simulink model "ESSSimulation"  (R2025a)
settings: Solver=VariableStepAuto  StartTime=0.0  StopTime=1800  RelTol=1e-3
undefined symbols (not defined in the file or in its folder): battery_builder_rtmsupport, gcbh
libraries: nesl_utility x18, P45B_98S30P_Library_lib x14, fl_lib x4, simulink x1, SignalEditorBlockLib x1
(part 3 of 8)

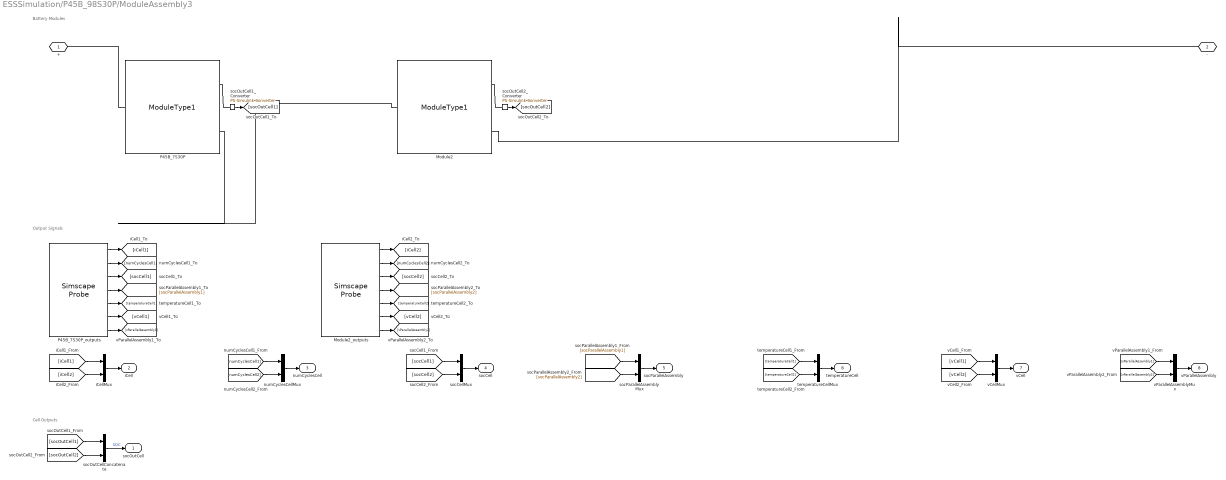
== system ESSSimulation/P45B_98S30P/ModuleAssembly3 ==
  note: Battery Modules
  note: Output Signals
  note: Cell Outputs
  Module2 : P45B_98S30P_Library_lib/Modules/ModuleType1  SOC_vecCell=[0, .01, .02, .03, .04, .05, .06, .07, .08, .09, .1, .11, .12, .13, .14, .15, .16, .17, .18, .19, .2, .21, .22, .23, .24, .25, .26, .27, .28, .29, .3, .31, .32, .33, .34, .35, .36, .37, .38, .39, .4, .41, .42, .43, .44, .45, .46, .47, .48, .49, .5, .51, .52, .53, .54, .55, .56, .57, .58, .59, .6, .61, .62, .63, .64, .65, .66, .67, .68, .69, .7, .71, .72, .73, .74, .75, .76, .77, .78, .79, .8, .81, .82, .83, .84, .85, .86, .87, .88, .89, .9, .91, .92, .93, .94, .95, .96, .97, .98, .99, 1]  T_vecCell=[-40, -30, -20, 0, 23, 45, 60] degC  V0_matCell=[3.17242, 3.17242, 3.17242, 3.17242, 3.17242, 3.17242, 3.17242; 3.18272, 3.18272, 3.18272, 3.18272, 3.18272, 3.18272, 3.18272; 3.19302, 3.19302, 3.19302, 3.19302, 3.19302, 3.19302, 3.19302; 3.20331, 3.20331, 3.20331, 3.20331, 3.20331, 3.20331, 3.20331; 3.21361, 3.21361, 3.21361, 3.21361, 3.21361, 3.21361, 3.21361; 3.22391, 3.22391, 3.22391, 3.22391, 3.22391, 3.22391, 3.22391; 3.23421, 3.23421, 3.23421, 3.23421, 3.23421, 3.23421, 3.23421; 3.24451, 3.24451, 3.24451, 3.24451, 3.24451, 3.24451, 3.24451; 3.25481, 3.25481, 3.25481, 3.25481, 3.25481, 3.25481, 3.25481; 3.2651, 3.2651, 3.2651, 3.2651, 3.2651, 3.2651, 3.2651; 3.2754, 3.2754, 3.2754, 3.2754, 3.2754, 3.2754, 3.2754; 3.2857, 3.2857, 3.2857, 3.2857, 3.2857, 3.2857, 3.2857; 3.296, 3.296, 3.296, 3.296, 3.296, 3.296, 3.296; 3.3063, 3.3063, 3.3063, 3.3063, 3.3063, 3.3063, 3.3063; 3.31659, 3.31659, 3.31659, 3.31659, 3.31659, 3.31659, 3.31659; 3.32689, 3.32689, 3.32689, 3.32689, 3.32689, 3.32689, 3.32689; 3.33719, 3.33719, 3.33719, 3.33719, 3.33719, 3.33719, 3.33719; 3.34749, 3.34749, 3.34749, 3.34749, 3.34749, 3.34749, 3.34749; 3.35779, 3.35779, 3.35779, 3.35779, 3.35779, 3.35779, 3.35779; 3.36809, 3.36809, 3.36809, 3.36809, 3.36809, 3.36809, 3.36809; 3.37838, 3.37838, 3.37838, 3.37838, 3.37838, 3.37838, 3.37838; 3.38868, 3.38868, 3.38868, 3.38868, 3.38868, 3.38868, 3.38868; 3.39898, 3.39898, 3.39898, 3.39898, 3.39898, 3.39898, 3.39898; 3.40928, 3.40928, 3.40928, 3.40928, 3.40928, 3.40928, 3.40928; 3.41958, 3.41958, 3.41958, 3.41958, 3.41958, 3.41958, 3.41958; 3.42988, 3.42988, 3.42988, 3.42988, 3.42988, 3.42988, 3.42988; 3.44017, 3.44017, 3.44017, 3.44017, 3.44017, 3.44017, 3.44017; 3.45047, 3.45047, 3.45047, 3.45047, 3.45047, 3.45047, 3.45047; 3.46077, 3.46077, 3.46077, 3.46077, 3.46077, 3.46077, 3.46077; 3.47107, 3.47107, 3.47107, 3.47107, 3.47107, 3.47107, 3.47107; 3.48137, 3.48137, 3.48137, 3.48137, 3.48137, 3.48137, 3.48137; 3.49166, 3.49166, 3.49166, 3.49166, 3.49166, 3.49166, 3.49166; 3.50196, 3.50196, 3.50196, 3.50196, 3.50196, 3.50196, 3.50196; 3.51226, 3.51226, 3.51226, 3.51226, 3.51226, 3.51226, 3.51226; 3.52256, 3.52256, 3.52256, 3.52256, 3.52256, 3.52256, 3.52256; 3.53286, 3.53286, 3.53286, 3.53286, 3.53286, 3.53286, 3.53286; 3.54316, 3.54316, 3.54316, 3.54316, 3.54316, 3.54316, 3.54316; 3.55345, 3.55345, 3.55345, 3.55345, 3.55345, 3.55345, 3.55345; 3.56375, 3.56375, 3.56375, 3.56375, 3.56375, 3.56375, 3.56375; 3.57405, 3.57405, 3.57405, 3.57405, 3.57405, 3.57405, 3.57405; 3.58435, 3.58435, 3.58435, 3.58435, 3.58435, 3.58435, 3.58435; 3.59465, 3.59465, 3.59465, 3.59465, 3.59465, 3.59465, 3.59465; 3.60495, 3.60495, 3.60495, 3.60495, 3.60495, 3.60495, 3.60495; 3.61524, 3.61524, 3.61524, 3.61524, 3.61524, 3.61524, 3.61524; 3.62554, 3.62554, 3.62554, 3.62554, 3.62554, 3.62554, 3.62554; 3.63584, 3.63584, 3.63584, 3.63584, 3.63584, 3.63584, 3.63584; 3.64614, 3.64614, 3.64614, 3.64614, 3.64614, 3.64614, 3.64614; 3.65644, 3.65644, 3.65644, 3.65644, 3.65644, 3.65644, 3.65644; 3.66673, 3.66673, 3.66673, 3.66673, 3.66673, 3.66673, 3.66673; 3.67703, 3.67703, 3.67703, 3.67703, 3.67703, 3.67703, 3.67703; 3.68733, 3.68733, 3.68733, 3.68733, 3.68733, 3.68733, 3.68733; 3.69763, 3.69763, 3.69763, 3.69763, 3.69763, 3.69763, 3.69763; 3.71041, 3.71041, 3.71041, 3.71041, 3.71041, 3.71041, 3.71041; 3.72113, 3.72113, 3.72113, 3.72113, 3.72113, 3.72113, 3.72113; 3.72997, 3.72997, 3.72997, 3.72997, 3.72997, 3.72997, 3.72997; 3.73882, 3.73882, 3.73882, 3.73882, 3.73882, 3.73882, 3.73882; 3.74912, 3.74912, 3.74912, 3.74912, 3.74912, 3.74912, 3.74912; 3.75936, 3.75936, 3.75936, 3.75936, 3.75936, 3.75936, 3.75936; 3.76951, 3.76951, 3.76951, 3.76951, 3.76951, 3.76951, 3.76951; 3.7791, 3.7791, 3.7791, 3.7791, 3.7791, 3.7791, 3.7791; 3.78865, 3.78865, 3.78865, 3.78865, 3.78865, 3.78865, 3.78865; 3.79787, 3.79787, 3.79787, 3.79787, 3.79787, 3.79787, 3.79787; 3.80709, 3.80709, 3.80709, 3.80709, 3.80709, 3.80709, 3.80709; 3.8161, 3.8161, 3.8161, 3.8161, 3.8161, 3.8161, 3.8161; 3.82509, 3.82509, ...(+2298 chars)] V  V_rangeCell=[2.25, Inf] V  R0_matCell=[.3026, .35142, .34349, .24415, .02095, .15874, .14729; .2941, .33555, .32379, .22614, .01921, .13363, .12249; .28559, .31969, .30408, .20813, .01774, .10853, .10276; .27709, .30382, .28438, .19012, .0166, .09423, .0861; .26858, .28796, .26468, .17211, .01557, .07998, .0748; .26008, .27209, .24498, .1541, .01469, .07024, .06679; .25157, .25623, .22527, .1361, .01398, .06387, .05877; .24307, .24036, .20557, .11861, .01338, .0575, .05275; .23456, .2245, .18587, .10674, .01283, .05113, .04899; .22606, .20863, .16617, .09525, .01239, .04679, .04522; .21755, .19277, .14651, .08799, .01196, .0439, .04145; .20905, .1769, .13098, .08073, .01155, .04101, .03817; .20054, .16103, .11905, .07347, .01116, .03813, .03522; .19204, .14769, .11102, .06895, .01079, .03524, .03228; .18353, .13913, .10517, .06499, .01042, .03235, .02934; .17503, .13157, .09933, .06104, .01007, .02946, .0264; .16653, .1271, .09371, .05708, .00974, .02657, .02345; .15804, .12264, .09094, .05312, .00949, .02417, .02125; .15354, .11817, .08816, .04917, .00924, .02286, .01972; .14976, .11385, .08539, .04748, .009, .02156, .0182; .14598, .11213, .08261, .04617, .00876, .02025, .01667; .14219, .11042, .08103, .04487, .00855, .01894, .01515; .14033, .10871, .08035, .04356, .00843, .01763, .01363; .13876, .10699, .07967, .04225, .00832, .01632, .0121; .13718, .10528, .07899, .04094, .00826, .01501, .01058; .13561, .10357, .07831, .03964, .00825, .0137, .00906; .13404, .10198, .07763, .03833, .00825, .01239, .00753; .13247, .10119, .07695, .03702, .00826, .01108, .0065; .13096, .10039, .07627, .03624, .00827, .00977, .00633; .13043, .0996, .07559, .03615, .00828, .00846, .00617; .1299, .0988, .07491, .03606, .0083, .00774, .006; .12937, .09801, .07423, .03597, .00834, .00779, .00583; .12883, .09721, .07355, .03588, .00838, .00783, .00567; .1283, .09642, .07301, .03579, .00842, .00787, .0055; .12777, .09585, .07296, .0357, .00848, .00792, .00534; .12724, .09584, .07291, .03561, .00855, .00796, .00517; .12675, .09584, .07286, .03552, .00863, .00801, .005; .12643, .09583, .0728, .03543, .00871, .00805, .00484; .12611, .09582, .07275, .03534, .00879, .00809, .00467; .12579, .09582, .0727, .03525, .00887, .00814, .0045; .12547, .09581, .07264, .03526, .00895, .00818, .00434; .12514, .0958, .07259, .03537, .00903, .00823, .00405; .12482, .09579, .07254, .03547, .00911, .00804, .00366; .1245, .09579, .07248, .03558, .00918, .00776, .00327; .12418, .09578, .07243, .03568, .00925, .00748, .00287; .12386, .09577, .07231, .03579, .00931, .0072, .00248; .12354, .09576, .0721, .03589, .00938, .00692, .00209; .12322, .09576, .07189, .036, .00946, .00664, .0017; .12301, .09575, .07168, .03611, .00953, .00636, .00131; .12309, .09574, .07147, .03621, .00961, .00608, .00092; .12318, .09573, .07125, .0363, .00968, .0058, .00053; .12326, .09573, .07104, .03637, .00976, .00552, .00014; .12389, .09628, .07138, .03699, .00991, .00579, .0003; .12407, .09637, .07126, .03715, .01, .0056, .0003; .12383, .09605, .07073, .0369, .01003, .00504, .0003; .12359, .09573, .07019, .03664, .01006, .00503, .0003; .12367, .09573, .06998, .03671, .01013, .00534, .00063; .12375, .09572, .06975, .03677, .01022, .00564, .00094; .1238, .09569, .07006, .0368, .0103, .00593, .00123; .12372, .09554, .07026, .03671, .01037, .00608, .00139; .12364, .09537, .07046, .03661, .01043, .00623, .00155; .12348, .09514, .07058, .03644, .01049, .0063, .00163; .12333, .0949, .07071, .03627, .01055, .00638, .00171; .12312, .09461, .07078, .03605, .01061, .00641, .00175; .12291, .09433, .07085, .03583, .01066, .00643, .00168; .12271, .09404, .07093, .03568, .01072, .00646, .00161; .12275, .09398, .071, .03622, .01077, .00646, .00153; .12316, .09449, .07107, .03677, .01082, .00636, .00145; .12357, .095, .07115, .03731, .01088, .00625, .00137; .12398, .09551, .07151, .03785, .01093, .00614, .00129; .12438, .09601, .07221, .03839, .01099, .00602, .0012; .12486, .09659, .07299, .039, .01105, .00599, .00119; .12548, .09731, .07391, ...(+1578 chars)] Ohm  AHCell=4.493 A*hr  extrapolation_optionCell=simscape.enum.extrapolation.nearest  thermal_massCell=63 J/K  P=30  S=7  iCell_specify=off  iCell_priority=None  iCell=0 A  iCell_nominal_specify=off  iCell_nominal_value=1  iCell_nominal_unit=A  vCell_specify=off  vCell_priority=None  vCell=0 V  vCell_nominal_specify=off  vCell_nominal_value=1  vCell_nominal_unit=V  socCell_specify=off  socCell_priority=High  socCell=1  socCell_nominal_specify=off  socCell_nominal_value=1  socCell_nominal_unit=1  numCyclesCell_specify=off  numCyclesCell_priority=High  numCyclesCell=0  numCyclesCell_nominal_specify=off  numCyclesCell_nominal_value=1  numCyclesCell_nominal_unit=1  temperatureCell_specify=off  temperatureCell_priority=High  temperatureCell=298.15 K  temperatureCell_nominal_specify=off  temperatureCell_nominal_value=1  temperatureCell_nominal_unit=K  vParallelAssembly_specify=off  vParallelAssembly_priority=None  vParallelAssembly=repmat(0, 7, 1) V  vParallelAssembly_nominal_specify=off  vParallelAssembly_nominal_value=1  vParallelAssembly_nominal_unit=V  socParallelAssembly_specify=off  socParallelAssembly_priority=None  socParallelAssembly=repmat(1, 7, 1)  socParallelAssembly_nominal_specify=off  socParallelAssembly_nominal_value=1  socParallelAssembly_nominal_unit=1
      settings: InternalSimscapePortConfiguration="{\"Bottom\":[{\"id\":\"n\",\"label\":\"-\",\"type\":\"foundation.electrical.electrical\"}],\"Left\":[],\"Right\":[{\"id\":\"socOutCell\",\"label\":\"SOC\",\"type\":\"output\"}],\"Top\":[{\"id\":\"p\",\"label\":\"+\",\"type\":\"foundation.electrical.electrical\"}]}"
  Module2_outputs : SimscapeProbe  BoundBlock=63  Variables="{\"iCell\":{\"Probing\":\"ON\"},\"numCyclesCell\":{\"Probing\":\"ON\"},\"socCell\":{\"Probing\":\"ON\"},\"socParallelAssembly\":{\"Probing\":\"ON\"},\"temperatureCell\":{\"Probing\":\"ON\"},\"vCell\":{\"Probing\":\"ON\"},\"vParallelAssembly\":{\"Probing\":\"ON\"}}"
  P45B_7S30P : P45B_98S30P_Library_lib/Modules/ModuleType1  SOC_vecCell=[0, .01, .02, .03, .04, .05, .06, .07, .08, .09, .1, .11, .12, .13, .14, .15, .16, .17, .18, .19, .2, .21, .22, .23, .24, .25, .26, .27, .28, .29, .3, .31, .32, .33, .34, .35, .36, .37, .38, .39, .4, .41, .42, .43, .44, .45, .46, .47, .48, .49, .5, .51, .52, .53, .54, .55, .56, .57, .58, .59, .6, .61, .62, .63, .64, .65, .66, .67, .68, .69, .7, .71, .72, .73, .74, .75, .76, .77, .78, .79, .8, .81, .82, .83, .84, .85, .86, .87, .88, .89, .9, .91, .92, .93, .94, .95, .96, .97, .98, .99, 1]  T_vecCell=[-40, -30, -20, 0, 23, 45, 60] degC  V0_matCell=[3.17242, 3.17242, 3.17242, 3.17242, 3.17242, 3.17242, 3.17242; 3.18272, 3.18272, 3.18272, 3.18272, 3.18272, 3.18272, 3.18272; 3.19302, 3.19302, 3.19302, 3.19302, 3.19302, 3.19302, 3.19302; 3.20331, 3.20331, 3.20331, 3.20331, 3.20331, 3.20331, 3.20331; 3.21361, 3.21361, 3.21361, 3.21361, 3.21361, 3.21361, 3.21361; 3.22391, 3.22391, 3.22391, 3.22391, 3.22391, 3.22391, 3.22391; 3.23421, 3.23421, 3.23421, 3.23421, 3.23421, 3.23421, 3.23421; 3.24451, 3.24451, 3.24451, 3.24451, 3.24451, 3.24451, 3.24451; 3.25481, 3.25481, 3.25481, 3.25481, 3.25481, 3.25481, 3.25481; 3.2651, 3.2651, 3.2651, 3.2651, 3.2651, 3.2651, 3.2651; 3.2754, 3.2754, 3.2754, 3.2754, 3.2754, 3.2754, 3.2754; 3.2857, 3.2857, 3.2857, 3.2857, 3.2857, 3.2857, 3.2857; 3.296, 3.296, 3.296, 3.296, 3.296, 3.296, 3.296; 3.3063, 3.3063, 3.3063, 3.3063, 3.3063, 3.3063, 3.3063; 3.31659, 3.31659, 3.31659, 3.31659, 3.31659, 3.31659, 3.31659; 3.32689, 3.32689, 3.32689, 3.32689, 3.32689, 3.32689, 3.32689; 3.33719, 3.33719, 3.33719, 3.33719, 3.33719, 3.33719, 3.33719; 3.34749, 3.34749, 3.34749, 3.34749, 3.34749, 3.34749, 3.34749; 3.35779, 3.35779, 3.35779, 3.35779, 3.35779, 3.35779, 3.35779; 3.36809, 3.36809, 3.36809, 3.36809, 3.36809, 3.36809, 3.36809; 3.37838, 3.37838, 3.37838, 3.37838, 3.37838, 3.37838, 3.37838; 3.38868, 3.38868, 3.38868, 3.38868, 3.38868, 3.38868, 3.38868; 3.39898, 3.39898, 3.39898, 3.39898, 3.39898, 3.39898, 3.39898; 3.40928, 3.40928, 3.40928, 3.40928, 3.40928, 3.40928, 3.40928; 3.41958, 3.41958, 3.41958, 3.41958, 3.41958, 3.41958, 3.41958; 3.42988, 3.42988, 3.42988, 3.42988, 3.42988, 3.42988, 3.42988; 3.44017, 3.44017, 3.44017, 3.44017, 3.44017, 3.44017, 3.44017; 3.45047, 3.45047, 3.45047, 3.45047, 3.45047, 3.45047, 3.45047; 3.46077, 3.46077, 3.46077, 3.46077, 3.46077, 3.46077, 3.46077; 3.47107, 3.47107, 3.47107, 3.47107, 3.47107, 3.47107, 3.47107; 3.48137, 3.48137, 3.48137, 3.48137, 3.48137, 3.48137, 3.48137; 3.49166, 3.49166, 3.49166, 3.49166, 3.49166, 3.49166, 3.49166; 3.50196, 3.50196, 3.50196, 3.50196, 3.50196, 3.50196, 3.50196; 3.51226, 3.51226, 3.51226, 3.51226, 3.51226, 3.51226, 3.51226; 3.52256, 3.52256, 3.52256, 3.52256, 3.52256, 3.52256, 3.52256; 3.53286, 3.53286, 3.53286, 3.53286, 3.53286, 3.53286, 3.53286; 3.54316, 3.54316, 3.54316, 3.54316, 3.54316, 3.54316, 3.54316; 3.55345, 3.55345, 3.55345, 3.55345, 3.55345, 3.55345, 3.55345; 3.56375, 3.56375, 3.56375, 3.56375, 3.56375, 3.56375, 3.56375; 3.57405, 3.57405, 3.57405, 3.57405, 3.57405, 3.57405, 3.57405; 3.58435, 3.58435, 3.58435, 3.58435, 3.58435, 3.58435, 3.58435; 3.59465, 3.59465, 3.59465, 3.59465, 3.59465, 3.59465, 3.59465; 3.60495, 3.60495, 3.60495, 3.60495, 3.60495, 3.60495, 3.60495; 3.61524, 3.61524, 3.61524, 3.61524, 3.61524, 3.61524, 3.61524; 3.62554, 3.62554, 3.62554, 3.62554, 3.62554, 3.62554, 3.62554; 3.63584, 3.63584, 3.63584, 3.63584, 3.63584, 3.63584, 3.63584; 3.64614, 3.64614, 3.64614, 3.64614, 3.64614, 3.64614, 3.64614; 3.65644, 3.65644, 3.65644, 3.65644, 3.65644, 3.65644, 3.65644; 3.66673, 3.66673, 3.66673, 3.66673, 3.66673, 3.66673, 3.66673; 3.67703, 3.67703, 3.67703, 3.67703, 3.67703, 3.67703, 3.67703; 3.68733, 3.68733, 3.68733, 3.68733, 3.68733, 3.68733, 3.68733; 3.69763, 3.69763, 3.69763, 3.69763, 3.69763, 3.69763, 3.69763; 3.71041, 3.71041, 3.71041, 3.71041, 3.71041, 3.71041, 3.71041; 3.72113, 3.72113, 3.72113, 3.72113, 3.72113, 3.72113, 3.72113; 3.72997, 3.72997, 3.72997, 3.72997, 3.72997, 3.72997, 3.72997; 3.73882, 3.73882, 3.73882, 3.73882, 3.73882, 3.73882, 3.73882; 3.74912, 3.74912, 3.74912, 3.74912, 3.74912, 3.74912, 3.74912; 3.75936, 3.75936, 3.75936, 3.75936, 3.75936, 3.75936, 3.75936; 3.76951, 3.76951, 3.76951, 3.76951, 3.76951, 3.76951, 3.76951; 3.7791, 3.7791, 3.7791, 3.7791, 3.7791, 3.7791, 3.7791; 3.78865, 3.78865, 3.78865, 3.78865, 3.78865, 3.78865, 3.78865; 3.79787, 3.79787, 3.79787, 3.79787, 3.79787, 3.79787, 3.79787; 3.80709, 3.80709, 3.80709, 3.80709, 3.80709, 3.80709, 3.80709; 3.8161, 3.8161, 3.8161, 3.8161, 3.8161, 3.8161, 3.8161; 3.82509, 3.82509, ...(+2298 chars)] V  V_rangeCell=[2.25, Inf] V  R0_matCell=[.3026, .35142, .34349, .24415, .02095, .15874, .14729; .2941, .33555, .32379, .22614, .01921, .13363, .12249; .28559, .31969, .30408, .20813, .01774, .10853, .10276; .27709, .30382, .28438, .19012, .0166, .09423, .0861; .26858, .28796, .26468, .17211, .01557, .07998, .0748; .26008, .27209, .24498, .1541, .01469, .07024, .06679; .25157, .25623, .22527, .1361, .01398, .06387, .05877; .24307, .24036, .20557, .11861, .01338, .0575, .05275; .23456, .2245, .18587, .10674, .01283, .05113, .04899; .22606, .20863, .16617, .09525, .01239, .04679, .04522; .21755, .19277, .14651, .08799, .01196, .0439, .04145; .20905, .1769, .13098, .08073, .01155, .04101, .03817; .20054, .16103, .11905, .07347, .01116, .03813, .03522; .19204, .14769, .11102, .06895, .01079, .03524, .03228; .18353, .13913, .10517, .06499, .01042, .03235, .02934; .17503, .13157, .09933, .06104, .01007, .02946, .0264; .16653, .1271, .09371, .05708, .00974, .02657, .02345; .15804, .12264, .09094, .05312, .00949, .02417, .02125; .15354, .11817, .08816, .04917, .00924, .02286, .01972; .14976, .11385, .08539, .04748, .009, .02156, .0182; .14598, .11213, .08261, .04617, .00876, .02025, .01667; .14219, .11042, .08103, .04487, .00855, .01894, .01515; .14033, .10871, .08035, .04356, .00843, .01763, .01363; .13876, .10699, .07967, .04225, .00832, .01632, .0121; .13718, .10528, .07899, .04094, .00826, .01501, .01058; .13561, .10357, .07831, .03964, .00825, .0137, .00906; .13404, .10198, .07763, .03833, .00825, .01239, .00753; .13247, .10119, .07695, .03702, .00826, .01108, .0065; .13096, .10039, .07627, .03624, .00827, .00977, .00633; .13043, .0996, .07559, .03615, .00828, .00846, .00617; .1299, .0988, .07491, .03606, .0083, .00774, .006; .12937, .09801, .07423, .03597, .00834, .00779, .00583; .12883, .09721, .07355, .03588, .00838, .00783, .00567; .1283, .09642, .07301, .03579, .00842, .00787, .0055; .12777, .09585, .07296, .0357, .00848, .00792, .00534; .12724, .09584, .07291, .03561, .00855, .00796, .00517; .12675, .09584, .07286, .03552, .00863, .00801, .005; .12643, .09583, .0728, .03543, .00871, .00805, .00484; .12611, .09582, .07275, .03534, .00879, .00809, .00467; .12579, .09582, .0727, .03525, .00887, .00814, .0045; .12547, .09581, .07264, .03526, .00895, .00818, .00434; .12514, .0958, .07259, .03537, .00903, .00823, .00405; .12482, .09579, .07254, .03547, .00911, .00804, .00366; .1245, .09579, .07248, .03558, .00918, .00776, .00327; .12418, .09578, .07243, .03568, .00925, .00748, .00287; .12386, .09577, .07231, .03579, .00931, .0072, .00248; .12354, .09576, .0721, .03589, .00938, .00692, .00209; .12322, .09576, .07189, .036, .00946, .00664, .0017; .12301, .09575, .07168, .03611, .00953, .00636, .00131; .12309, .09574, .07147, .03621, .00961, .00608, .00092; .12318, .09573, .07125, .0363, .00968, .0058, .00053; .12326, .09573, .07104, .03637, .00976, .00552, .00014; .12389, .09628, .07138, .03699, .00991, .00579, .0003; .12407, .09637, .07126, .03715, .01, .0056, .0003; .12383, .09605, .07073, .0369, .01003, .00504, .0003; .12359, .09573, .07019, .03664, .01006, .00503, .0003; .12367, .09573, .06998, .03671, .01013, .00534, .00063; .12375, .09572, .06975, .03677, .01022, .00564, .00094; .1238, .09569, .07006, .0368, .0103, .00593, .00123; .12372, .09554, .07026, .03671, .01037, .00608, .00139; .12364, .09537, .07046, .03661, .01043, .00623, .00155; .12348, .09514, .07058, .03644, .01049, .0063, .00163; .12333, .0949, .07071, .03627, .01055, .00638, .00171; .12312, .09461, .07078, .03605, .01061, .00641, .00175; .12291, .09433, .07085, .03583, .01066, .00643, .00168; .12271, .09404, .07093, .03568, .01072, .00646, .00161; .12275, .09398, .071, .03622, .01077, .00646, .00153; .12316, .09449, .07107, .03677, .01082, .00636, .00145; .12357, .095, .07115, .03731, .01088, .00625, .00137; .12398, .09551, .07151, .03785, .01093, .00614, .00129; .12438, .09601, .07221, .03839, .01099, .00602, .0012; .12486, .09659, .07299, .039, .01105, .00599, .00119; .12548, .09731, .07391, ...(+1578 chars)] Ohm  AHCell=4.493 A*hr  extrapolation_optionCell=simscape.enum.extrapolation.nearest  thermal_massCell=63 J/K  P=30  S=7  iCell_specify=off  iCell_priority=None  iCell=0 A  iCell_nominal_specify=off  iCell_nominal_value=1  iCell_nominal_unit=A  vCell_specify=off  vCell_priority=None  vCell=0 V  vCell_nominal_specify=off  vCell_nominal_value=1  vCell_nominal_unit=V  socCell_specify=off  socCell_priority=High  socCell=1  socCell_nominal_specify=off  socCell_nominal_value=1  socCell_nominal_unit=1  numCyclesCell_specify=off  numCyclesCell_priority=High  numCyclesCell=0  numCyclesCell_nominal_specify=off  numCyclesCell_nominal_value=1  numCyclesCell_nominal_unit=1  temperatureCell_specify=off  temperatureCell_priority=High  temperatureCell=298.15 K  temperatureCell_nominal_specify=off  temperatureCell_nominal_value=1  temperatureCell_nominal_unit=K  vParallelAssembly_specify=off  vParallelAssembly_priority=None  vParallelAssembly=repmat(0, 7, 1) V  vParallelAssembly_nominal_specify=off  vParallelAssembly_nominal_value=1  vParallelAssembly_nominal_unit=V  socParallelAssembly_specify=off  socParallelAssembly_priority=None  socParallelAssembly=repmat(1, 7, 1)  socParallelAssembly_nominal_specify=off  socParallelAssembly_nominal_value=1  socParallelAssembly_nominal_unit=1
      settings: InternalSimscapePortConfiguration="{\"Bottom\":[{\"id\":\"n\",\"label\":\"-\",\"type\":\"foundation.electrical.electrical\"}],\"Left\":[],\"Right\":[{\"id\":\"socOutCell\",\"label\":\"SOC\",\"type\":\"output\"}],\"Top\":[{\"id\":\"p\",\"label\":\"+\",\"type\":\"foundation.electrical.electrical\"}]}"
  P45B_7S30P_outputs : SimscapeProbe  BoundBlock=65  Variables="{\"iCell\":{\"Probing\":\"ON\"},\"numCyclesCell\":{\"Probing\":\"ON\"},\"socCell\":{\"Probing\":\"ON\"},\"socParallelAssembly\":{\"Probing\":\"ON\"},\"temperatureCell\":{\"Probing\":\"ON\"},\"vCell\":{\"Probing\":\"ON\"},\"vParallelAssembly\":{\"Probing\":\"ON\"}}"
  iCellMux : Mux  Inputs=2
  numCyclesCellMux : Mux  Inputs=2
  socCellMux : Mux  Inputs=2
  socOutCell1_Converter : nesl_utility/PS-Simulink Converter  PhysicalDomain=network_engine_domain  SubClassName=ps_output  LeftPortType=input  RightPortType=output  PseudoPeriodic=off  Frequencies=[]  VectorFormat=inherit  Unit=inherit  AffineConversion=off
  socOutCell2_Converter : nesl_utility/PS-Simulink Converter  PhysicalDomain=network_engine_domain  SubClassName=ps_output  LeftPortType=input  RightPortType=output  PseudoPeriodic=off  Frequencies=[]  VectorFormat=inherit  Unit=inherit  AffineConversion=off
  socOutCellConcatenate : Concatenate  Mode=Multidimensional array  ConcatenateDimension=2
  socParallelAssemblyMux : Mux  Inputs=2
  temperatureCellMux : Mux  Inputs=2
  vCellMux : Mux  Inputs=2
  vParallelAssemblyMux : Mux  Inputs=2
  + : PMIOPort  Side=Left
  - : PMIOPort  Port=2  Side=Right
  socOutCell : Outport
  iCell : Outport  Port=2
  numCyclesCell : Outport  Port=3
  socCell : Outport  Port=4
  socParallelAssembly : Outport  Port=5
  temperatureCell : Outport  Port=6
  vCell : Outport  Port=7
  vParallelAssembly : Outport  Port=8
  wires:
  socOutCellConcatenate/1 -> socOutCell/1  "SOC"
  [socOutCell1] -> socOutCellConcatenate/1
  [socOutCell2] -> socOutCellConcatenate/2
  P45B_7S30P_outputs/1 -> [iCell1]
  iCellMux/1 -> iCell/1
  [iCell1] -> iCellMux/1
  P45B_7S30P_outputs/2 -> [numCyclesCell1]
  numCyclesCellMux/1 -> numCyclesCell/1
  [numCyclesCell1] -> numCyclesCellMux/1
  P45B_7S30P_outputs/3 -> [socCell1]
  socCellMux/1 -> socCell/1
  [socCell1] -> socCellMux/1
  P45B_7S30P_outputs/4 -> [socParallelAssembly1]
  socParallelAssemblyMux/1 -> socParallelAssembly/1
  [socParallelAssembly1] -> socParallelAssemblyMux/1
  P45B_7S30P_outputs/5 -> [temperatureCell1]
  temperatureCellMux/1 -> temperatureCell/1
  [temperatureCell1] -> temperatureCellMux/1
  P45B_7S30P_outputs/6 -> [vCell1]
  vCellMux/1 -> vCell/1
  [vCell1] -> vCellMux/1
  P45B_7S30P_outputs/7 -> [vParallelAssembly1]
  vParallelAssemblyMux/1 -> vParallelAssembly/1
  [vParallelAssembly1] -> vParallelAssemblyMux/1
  Module2_outputs/1 -> [iCell2]
  [iCell2] -> iCellMux/2
  Module2_outputs/2 -> [numCyclesCell2]
  [numCyclesCell2] -> numCyclesCellMux/2
  Module2_outputs/3 -> [socCell2]
  [socCell2] -> socCellMux/2
  Module2_outputs/4 -> [socParallelAssembly2]
  [socParallelAssembly2] -> socParallelAssemblyMux/2
  Module2_outputs/5 -> [temperatureCell2]
  [temperatureCell2] -> temperatureCellMux/2
  Module2_outputs/6 -> [vCell2]
  [vCell2] -> vCellMux/2
  Module2_outputs/7 -> [vParallelAssembly2]
  [vParallelAssembly2] -> vParallelAssemblyMux/2
  socOutCell1_Converter/1 -> [socOutCell1]
  socOutCell2_Converter/1 -> [socOutCell2]
  connections:
  Module2/LConn1 -- P45B_7S30P/RConn2
  P45B_7S30P/LConn1 -- +/RConn1
  Module2/RConn2 -- -/RConn1
  socOutCell1_Converter/LConn1 -- P45B_7S30P/RConn1
  socOutCell2_Converter/LConn1 -- Module2/RConn1
